simulink model "W06_1_point"  (R2024b)
settings: Solver=ode4  StartTime=0.0  StopTime=T_run  FixedStep=Ts_ctrl  RelTol=1e-3
InitFcn:
  | if ~exist('W06_model_init','file'), addpath(fileparts(get_param('W06_1_point','FileName'))); end, W06_model_init('W06_1_point')
StopFcn:
  | W06_model_done('W06_1_point')
values from neighbouring files (symbols this model uses):
  alloc_prm = [half_beam; l_bow; F_max; F_bow_max]    [W06_setup.m]
  animate = 0    [W06_bow_demo.m]    (also in W06_psi_sweep.m; W06_setup.m = 1)
  beta_c = deg2rad(current_direction)    [W06_setup.m]
  current_speed = 0.0    (= 0)    [W06_setup.m]
  F_bow_max = 250    [W06_setup.m]
  F_max = 500    [W06_setup.m]
  half_beam = 1.027135    [W06_setup.m]
  Kb = Ki_u / Kp_u    (= 0.333333333333)    [W06_setup.m]
  Kd_psi = 200    [W06_setup.m]
  Ki_u = 100    [W06_setup.m]
  Ki_v = 100    [W06_setup.m]
  Kp_psi = 400    [W06_setup.m]
  Kp_u = 300    [W06_setup.m]
  Kp_v = 300    [W06_setup.m]
  Kp_x = 0.4    [W06_setup.m]
  Kp_y = 0.4    [W06_setup.m]
  l_bow = 0.75    [W06_setup.m]
  psi_d = deg2rad(PSI(i))    [W06_psi_sweep.m]    (also in W06_setup.m = deg2rad(hold_deg))
  Ts_ctrl = 0.05    [W06_setup.m]
  u_max = 1.5    [W06_setup.m]
  usv_p = [m_usv; Izz; Xu; Xuu; Yv; Yvv; Nr; Nrr; half_beam; l_bow]    [W06_setup.m]
  v_max = 0.6    [W06_setup.m]
  x0 = [0.1; 0; 0; 0; 0; psi_init]    [W06_setup.m]
  x_d = hold_north    (= 30)    [W06_setup.m]
  y_d = hold_east    (= 20)    [W06_setup.m]
libraries: slpidlib x2
settings Model: Creator=admin  LastModifiedBy=admin

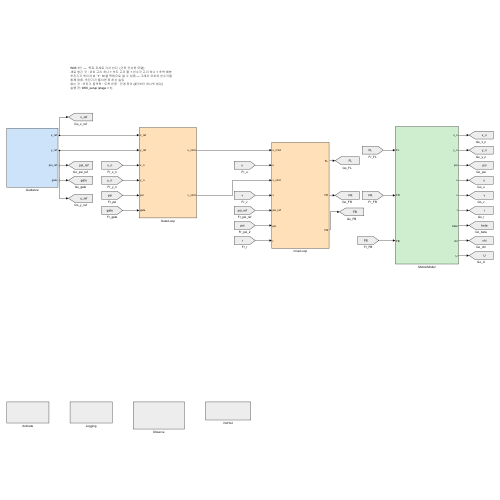
[thumbnail: Simulink's stored preview of the top-level diagram]
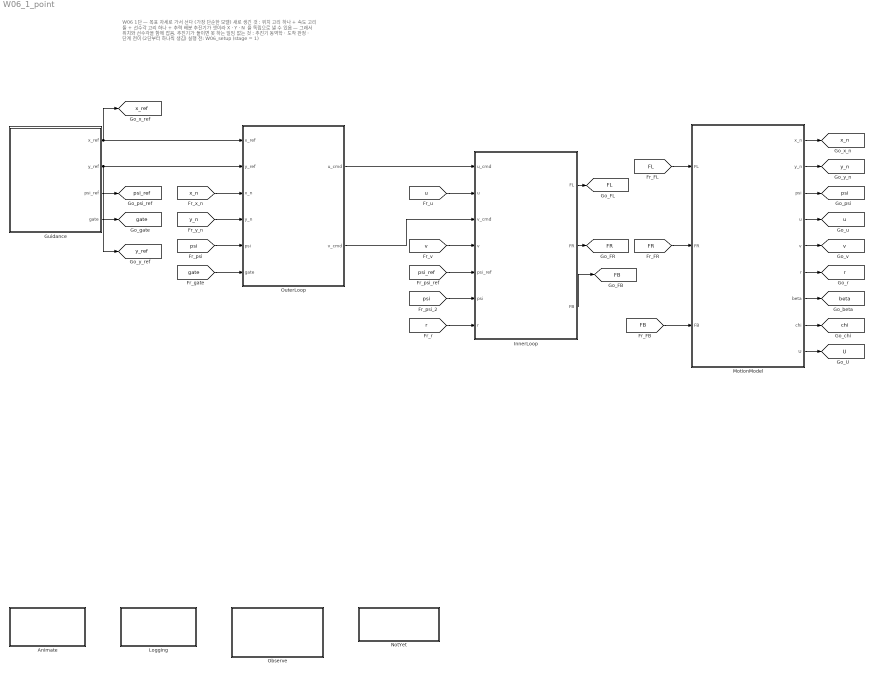
== system W06_1_point ==
  note: W06 1단  —  목표 자세로 가서 선다  (가장 단순한 모델)
      | 새로 생긴 것 : 위치 고리 하나 + 속도 고리 둘 + 선수각 고리 하나 + 추력 배분
      | 추진기가 셋이라 X · Y · N 을 독립으로 낼 수 있음 — 그래서 위치와 선수각을
      | 함께 잡음. 추진기가 둘이면 못 하는 일임
      | 없는 것 : 추진기 동역학 · 도착 판정 · 단계 전이 (2단부터 하나씩 생김)
      | 실행 전: W06_setup (stage = 1)
  Animate : Subsystem
  Guidance : Subsystem
  InnerLoop : Subsystem
  Logging : Subsystem
  MotionModel : Subsystem
  NotYet : Subsystem
  Observe : Subsystem
  OuterLoop : Subsystem
  tag scope: FB=global, FL=global, FR=global, U=global, beta=global, chi=global, gate=global, psi=global, psi_ref=global, r=global, u=global, v=global, x_n=global, x_ref=global, y_n=global, y_ref=global
  wires:
  OuterLoop/2(v_cmd) -> InnerLoop/3(v_cmd)
  OuterLoop/1(u_cmd) -> InnerLoop/1(u_cmd)
  Guidance/1(x_ref) -> OuterLoop/1(x_ref), [x_ref]
  Guidance/2(y_ref) -> OuterLoop/2(y_ref), [y_ref]
  MotionModel/3(psi) -> [psi]
  Guidance/3(psi_ref) -> [psi_ref]
  MotionModel/6(r) -> [r]
  MotionModel/4(u) -> [u]
  MotionModel/5(v) -> [v]
  MotionModel/1(x_n) -> [x_n]
  MotionModel/2(y_n) -> [y_n]
  [FB] -> MotionModel/3(FB)
  [psi] -> InnerLoop/6(psi)
  [psi_ref] -> InnerLoop/5(psi_ref)
  [r] -> InnerLoop/7(r)
  [u] -> InnerLoop/2(u)
  [v] -> InnerLoop/4(v)
  [x_n] -> OuterLoop/3(x_n)
  [y_n] -> OuterLoop/4(y_n)
  MotionModel/9(U) -> [U]
  MotionModel/7(beta) -> [beta]
  MotionModel/8(chi) -> [chi]
  Guidance/4(gate) -> [gate]
  [psi] -> OuterLoop/5(psi)
  [gate] -> OuterLoop/6(gate)
  InnerLoop/3(FB) -> [FB]
  InnerLoop/1(FL) -> [FL]
  InnerLoop/2(FR) -> [FR]
  [FL] -> MotionModel/1(FL)
  [FR] -> MotionModel/2(FR)

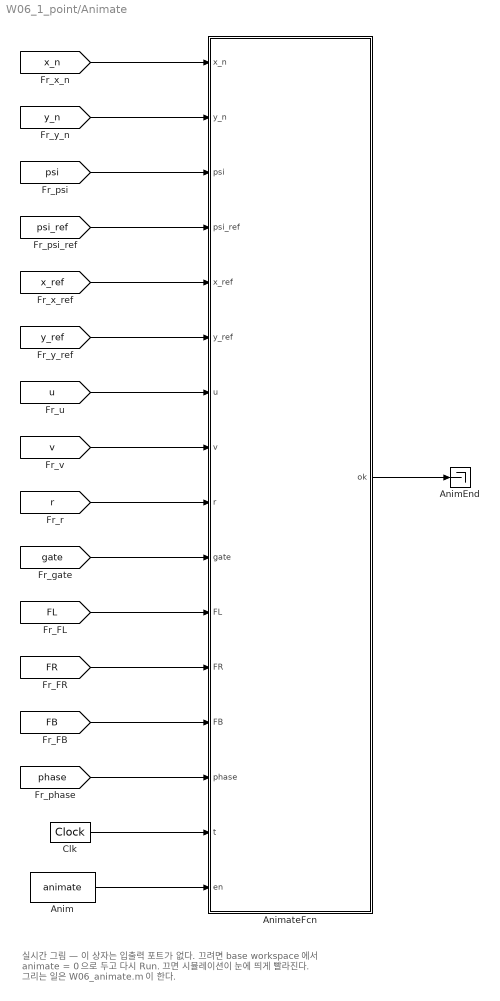
== system W06_1_point/Animate ==
  note: 실시간 그림 — 이 상자는 입출력 포트가 없다.
      | 끄려면 base workspace 에서  animate = 0  으로 두고 다시 Run.
      | 끄면 시뮬레이션이 눈에 띄게 빨라진다.
      | 그리는 일은 W06_animate.m 이 한다.
  Anim : Constant  Value=animate
  AnimEnd : Terminator
  AnimateFcn : MATLAB Function  TreatAsAtomicUnit=on
  Clk : DigitalClock  SampleTime=Ts_ctrl
  wires:
  [x_n] -> AnimateFcn/1(x_n)
  [y_n] -> AnimateFcn/2(y_n)
  [psi] -> AnimateFcn/3(psi)
  [psi_ref] -> AnimateFcn/4(psi_ref)
  [x_ref] -> AnimateFcn/5(x_ref)
  [y_ref] -> AnimateFcn/6(y_ref)
  [u] -> AnimateFcn/7(u)
  [v] -> AnimateFcn/8(v)
  [r] -> AnimateFcn/9(r)
  [gate] -> AnimateFcn/10(gate)
  [FL] -> AnimateFcn/11(FL)
  [FR] -> AnimateFcn/12(FR)
  [FB] -> AnimateFcn/13(FB)
  [phase] -> AnimateFcn/14(phase)
  Clk/1 -> AnimateFcn/15(t)
  Anim/1 -> AnimateFcn/16(en)
  AnimateFcn/1(ok) -> AnimEnd/1

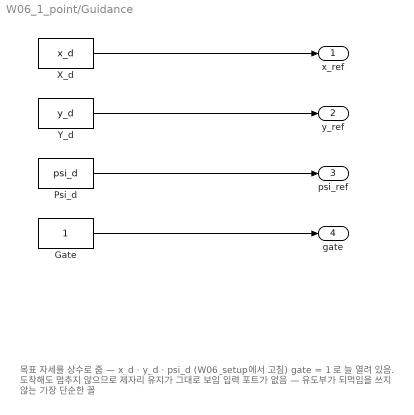
== system W06_1_point/Guidance ==
  note: 목표 자세를 상수로 줌 — x_d · y_d · psi_d (W06_setup 에서 고침)
      | gate = 1 로 늘 열려 있음. 도착해도 멈추지 않으므로 제자리 유지가 그대로 보임
      | 입력 포트가 없음 — 유도부가 되먹임을 쓰지 않는 가장 단순한 꼴
  Gate : Constant
  Psi_d : Constant  Value=psi_d
  X_d : Constant  Value=x_d
  Y_d : Constant  Value=y_d
  x_ref : Outport
  y_ref : Outport  Port=2
  psi_ref : Outport  Port=3
  gate : Outport  Port=4
  wires:
  X_d/1 -> x_ref/1
  Y_d/1 -> y_ref/1
  Psi_d/1 -> psi_ref/1
  Gate/1 -> gate/1

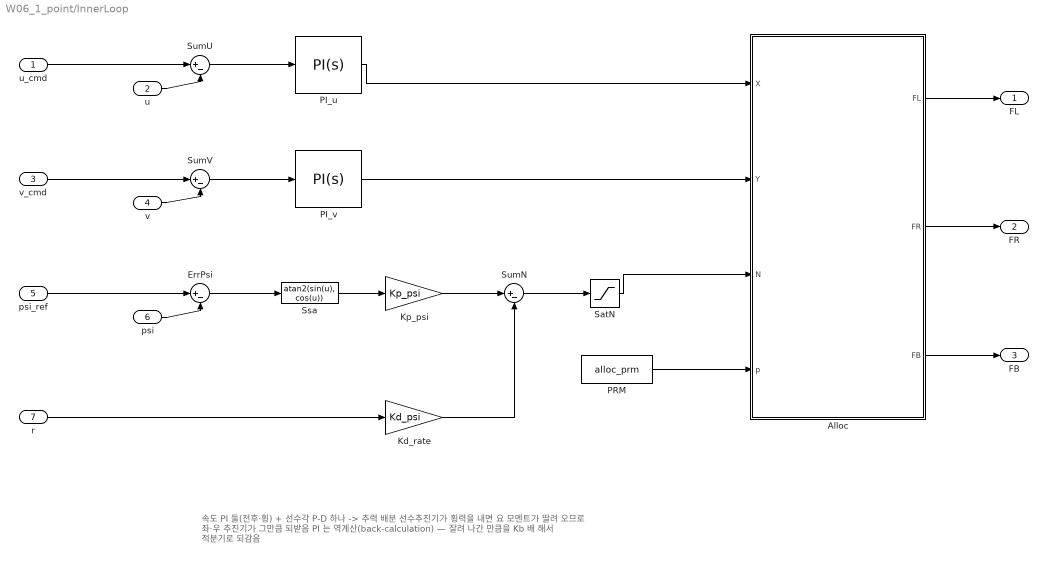
== system W06_1_point/InnerLoop ==
  note: 속도 PI 둘(전후·횡) + 선수각 P-D 하나 -> 추력 배분
      | 선수추진기가 횡력을 내면 요 모멘트가 딸려 오므로 좌·우 추진기가 그만큼 되받음
      | PI 는 역계산(back-calculation) — 잘려 나간 만큼을 Kb 배 해서 적분기로 되감음
  u_cmd : Inport
  u : Inport  Port=2
  v_cmd : Inport  Port=3
  v : Inport  Port=4
  psi_ref : Inport  Port=5
  psi : Inport  Port=6
  r : Inport  Port=7
  Alloc : MATLAB Function  TreatAsAtomicUnit=on
  ErrPsi : Sum  Inputs=|+-
  Kd_rate : Gain  Gain=Kd_psi
  Kp_psi : Gain  Gain=Kp_psi
  PI_u : slpidlib/PID Controller  Controller=PI  Form=Parallel  TimeDomain=Continuous-time  UseExternalTs=off  SampleTime=-1  IntegratorMethod=Forward Euler  FilterMethod=Forward Euler  ControllerParametersSource=internal  P=Kp_u  I=Ki_u  UseKiTs=off  D=0  UseExternalDerivativeSource=off  N=100  UseFilter=on  TunerSelectOption=Transfer Function Based (PID Tuner App)  InitialConditionSource=internal  InitialConditionForIntegrator=0  InitialConditionForFilter=0  DifferentiatorICPrevScaledInput=0  ExternalReset=none  TrackingMode=off  Kt=1  LimitOutput=on  SatLimitsSource=internal  UpperSaturationLimit=2*F_max  LowerSaturationLimit=-(2*F_max)  LinearizeAsGain=on  AntiWindupMode=back-calculation  Kb=Kb  LimitIntegrator=off  UpperIntegratorSaturationLimit=inf  LowerIntegratorSaturationLimit=-inf  POutMin=[]  POutMax=[]  IOutMin=[]  IOutMax=[]  DOutMin=[]  DOutMax=[]  NOutMin=[]  NOutMax=[]  SumOutMin=[]  SumOutMax=[]  SaturationOutMin=[]  SaturationOutMax=[]  PParamMin=[]  PParamMax=[]  IParamMin=[]  IParamMax=[]  DParamMin=[]  DParamMax=[]  NParamMin=[]  NParamMax=[]  KbParamMin=[]  KbParamMax=[]  KtParamMin=[]  KtParamMax=[]  KbOutMin=[]  KbOutMax=[]  KtOutMin=[]  KtOutMax=[]  IntegratorOutMin=[]  IntegratorOutMax=[]  FilterOutMin=[]  FilterOutMax=[]  SumI1OutMin=[]  SumI1OutMax=[]  SumI2OutMin=[]  SumI2OutMax=[]  SumI3OutMin=[]  SumI3OutMax=[]  SumI4OutMin=[]  SumI4OutMax=[]  SumDOutMin=[]  SumDOutMax=[]  DifferentiatorOutMin=[]  DifferentiatorOutMax=[]  FilterDiffOutCoefMin=[]  FilterDiffOutCoefMax=[]  ReciprocalOutMin=[]  ReciprocalOutMax=[]  SumDenOutMin=[]  SumDenOutMax=[]  SumNumOutMin=[]  SumNumOutMax=[]  DivideOutMin=[]  DivideOutMax=[]  UdiffTsProdOutMin=[]  UdiffTsProdOutMax=[]  NTsProdOutMin=[]  NTsProdOutMax=[]  UintegralTsProdOutMin=[]  UintegralTsProdOutMax=[]  UngainTsProdOutMin=[]  UngainTsProdOutMax=[]  ClampingZeroOutDataTypeStr=Inherit: Inherit via back propagation  ClampingZeroOutMin=[]  ClampingZeroOutMax=[]  FilterDenConstantOutDataTypeStr=Inherit: Inherit via back propagation  FilterDenConstantOutMin=[]  FilterDenConstantOutMax=[]  PCopyOutDataTypeStr=Inherit: Inherit via back propagation  PCopyOutMin=[]  PCopyOutMax=[]  NCopyOutDataTypeStr=Inherit: Inherit via back propagation  NCopyOutMin=[]  NCopyOutMax=[]  IntegratorContinuousStateAttributes=''  IntegratorStateMustResolveToSignalObject=off  IntegratorRTWStateStorageClass=Auto  FilterContinuousStateAttributes=''  FilterStateMustResolveToSignalObject=off  FilterRTWStateStorageClass=Auto  ParallelPVariant=InternalParameters  IdealPVariant=Disabled  IVariant=InternalParameters  DVariant=Disabled  IntegratorVariant=Continuous  SatVariant=Enabled  AWVariant=BackCalculation  PCopyVariant=Disabled  TRVariant=Disabled  FdbkBlocksVariant=Forward  IdealPFdbkVariant=Disabled  SatFdbkVariant=Disabled  DerivativeFilterVariant=Disabled  NVariant=Disabled  NCopyVariant=Disabled_SignalSpec  FilterICVariant=Disabled  IntegratorICVariant=InternalICs  ExternalResetVariant=Disabled  TRSumVariant=Passthrough  SumFdbkVariant=Disabled  SumVariant=Sum_PI  TsampFilterVariant=InternalTs  TsampNgainVariant=Passthrough  TsampIntegralVariant=Disabled_SignalSpec  ExternalSaturationOutDataTypeStr=Inherit: Same as second input  DerivativeSourceVariant=Disabled  PreIntVariant=InternalPreInt
  PI_v : slpidlib/PID Controller  Controller=PI  Form=Parallel  TimeDomain=Continuous-time  UseExternalTs=off  SampleTime=-1  IntegratorMethod=Forward Euler  FilterMethod=Forward Euler  ControllerParametersSource=internal  P=Kp_v  I=Ki_v  UseKiTs=off  D=0  UseExternalDerivativeSource=off  N=100  UseFilter=on  TunerSelectOption=Transfer Function Based (PID Tuner App)  InitialConditionSource=internal  InitialConditionForIntegrator=0  InitialConditionForFilter=0  DifferentiatorICPrevScaledInput=0  ExternalReset=none  TrackingMode=off  Kt=1  LimitOutput=on  SatLimitsSource=internal  UpperSaturationLimit=F_bow_max  LowerSaturationLimit=-(F_bow_max)  LinearizeAsGain=on  AntiWindupMode=back-calculation  Kb=Kb  LimitIntegrator=off  UpperIntegratorSaturationLimit=inf  LowerIntegratorSaturationLimit=-inf  POutMin=[]  POutMax=[]  IOutMin=[]  IOutMax=[]  DOutMin=[]  DOutMax=[]  NOutMin=[]  NOutMax=[]  SumOutMin=[]  SumOutMax=[]  SaturationOutMin=[]  SaturationOutMax=[]  PParamMin=[]  PParamMax=[]  IParamMin=[]  IParamMax=[]  DParamMin=[]  DParamMax=[]  NParamMin=[]  NParamMax=[]  KbParamMin=[]  KbParamMax=[]  KtParamMin=[]  KtParamMax=[]  KbOutMin=[]  KbOutMax=[]  KtOutMin=[]  KtOutMax=[]  IntegratorOutMin=[]  IntegratorOutMax=[]  FilterOutMin=[]  FilterOutMax=[]  SumI1OutMin=[]  SumI1OutMax=[]  SumI2OutMin=[]  SumI2OutMax=[]  SumI3OutMin=[]  SumI3OutMax=[]  SumI4OutMin=[]  SumI4OutMax=[]  SumDOutMin=[]  SumDOutMax=[]  DifferentiatorOutMin=[]  DifferentiatorOutMax=[]  FilterDiffOutCoefMin=[]  FilterDiffOutCoefMax=[]  ReciprocalOutMin=[]  ReciprocalOutMax=[]  SumDenOutMin=[]  SumDenOutMax=[]  SumNumOutMin=[]  SumNumOutMax=[]  DivideOutMin=[]  DivideOutMax=[]  UdiffTsProdOutMin=[]  UdiffTsProdOutMax=[]  NTsProdOutMin=[]  NTsProdOutMax=[]  UintegralTsProdOutMin=[]  UintegralTsProdOutMax=[]  UngainTsProdOutMin=[]  UngainTsProdOutMax=[]  ClampingZeroOutDataTypeStr=Inherit: Inherit via back propagation  ClampingZeroOutMin=[]  ClampingZeroOutMax=[]  FilterDenConstantOutDataTypeStr=Inherit: Inherit via back propagation  FilterDenConstantOutMin=[]  FilterDenConstantOutMax=[]  PCopyOutDataTypeStr=Inherit: Inherit via back propagation  PCopyOutMin=[]  PCopyOutMax=[]  NCopyOutDataTypeStr=Inherit: Inherit via back propagation  NCopyOutMin=[]  NCopyOutMax=[]  IntegratorContinuousStateAttributes=''  IntegratorStateMustResolveToSignalObject=off  IntegratorRTWStateStorageClass=Auto  FilterContinuousStateAttributes=''  FilterStateMustResolveToSignalObject=off  FilterRTWStateStorageClass=Auto  ParallelPVariant=InternalParameters  IdealPVariant=Disabled  IVariant=InternalParameters  DVariant=Disabled  IntegratorVariant=Continuous  SatVariant=Enabled  AWVariant=BackCalculation  PCopyVariant=Disabled  TRVariant=Disabled  FdbkBlocksVariant=Forward  IdealPFdbkVariant=Disabled  SatFdbkVariant=Disabled  DerivativeFilterVariant=Disabled  NVariant=Disabled  NCopyVariant=Disabled_SignalSpec  FilterICVariant=Disabled  IntegratorICVariant=InternalICs  ExternalResetVariant=Disabled  TRSumVariant=Passthrough  SumFdbkVariant=Disabled  SumVariant=Sum_PI  TsampFilterVariant=InternalTs  TsampNgainVariant=Passthrough  TsampIntegralVariant=Disabled_SignalSpec  ExternalSaturationOutDataTypeStr=Inherit: Same as second input  DerivativeSourceVariant=Disabled  PreIntVariant=InternalPreInt
  PRM : Constant  Value=alloc_prm
  SatN : Saturate  UpperLimit=2*F_max*half_beam + F_bow_max*l_bow  LowerLimit=-(2*F_max*half_beam + F_bow_max*l_bow)
  Ssa : Fcn  Expr=atan2(sin(u), cos(u))
  SumN : Sum  Inputs=|+-
  SumU : Sum  Inputs=|+-
  SumV : Sum  Inputs=|+-
  FL : Outport
  FR : Outport  Port=2
  FB : Outport  Port=3
  wires:
  u_cmd/1 -> SumU/1
  u/1 -> SumU/2
  v_cmd/1 -> SumV/1
  v/1 -> SumV/2
  SumU/1 -> PI_u/1
  SumV/1 -> PI_v/1
  ErrPsi/1 -> Ssa/1
  psi_ref/1 -> ErrPsi/1
  psi/1 -> ErrPsi/2
  Ssa/1 -> Kp_psi/1
  r/1 -> Kd_rate/1
  Kp_psi/1 -> SumN/1
  Kd_rate/1 -> SumN/2
  SumN/1 -> SatN/1
  PI_u/1 -> Alloc/1(X)
  PI_v/1 -> Alloc/2(Y)
  SatN/1 -> Alloc/3(N)
  PRM/1 -> Alloc/4(p)
  Alloc/1(FL) -> FL/1
  Alloc/2(FR) -> FR/1
  Alloc/3(FB) -> FB/1

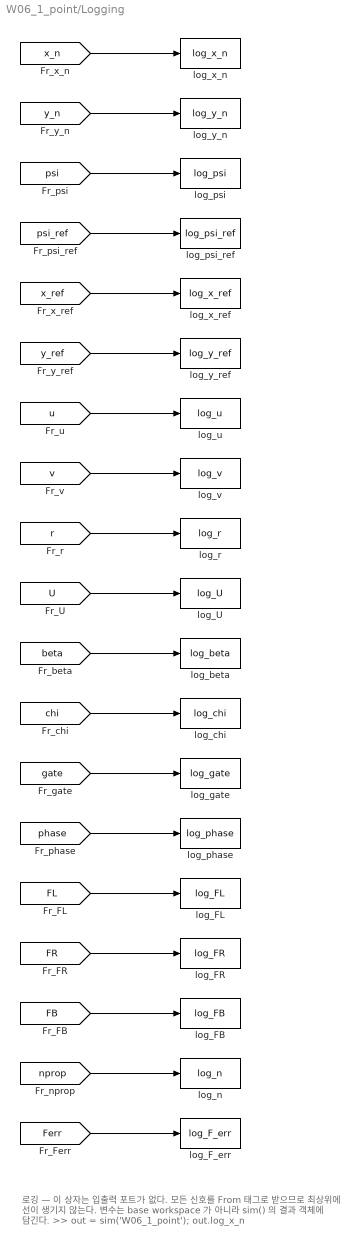
== system W06_1_point/Logging ==
  note: 로깅 — 이 상자는 입출력 포트가 없다.
      | 모든 신호를 From 태그로 받으므로 최상위에 선이 생기지 않는다.
      | 변수는 base workspace 가 아니라 sim() 의 결과 객체에 담긴다.
      |   >> out = sim('W06_1_point');  out.log_x_n
  log_FB : ToWorkspace  VariableName=log_FB  SaveFormat=Timeseries  SampleTime=Ts_ctrl
  log_FL : ToWorkspace  VariableName=log_FL  SaveFormat=Timeseries  SampleTime=Ts_ctrl
  log_FR : ToWorkspace  VariableName=log_FR  SaveFormat=Timeseries  SampleTime=Ts_ctrl
  log_F_err : ToWorkspace  VariableName=log_F_err  SaveFormat=Timeseries  SampleTime=Ts_ctrl
  log_U : ToWorkspace  VariableName=log_U  SaveFormat=Timeseries  SampleTime=Ts_ctrl
  log_beta : ToWorkspace  VariableName=log_beta  SaveFormat=Timeseries  SampleTime=Ts_ctrl
  log_chi : ToWorkspace  VariableName=log_chi  SaveFormat=Timeseries  SampleTime=Ts_ctrl
  log_gate : ToWorkspace  VariableName=log_gate  SaveFormat=Timeseries  SampleTime=Ts_ctrl
  log_n : ToWorkspace  VariableName=log_n  SaveFormat=Timeseries  SampleTime=Ts_ctrl
  log_phase : ToWorkspace  VariableName=log_phase  SaveFormat=Timeseries  SampleTime=Ts_ctrl
  log_psi : ToWorkspace  VariableName=log_psi  SaveFormat=Timeseries  SampleTime=Ts_ctrl
  log_psi_ref : ToWorkspace  VariableName=log_psi_ref  SaveFormat=Timeseries  SampleTime=Ts_ctrl
  log_r : ToWorkspace  VariableName=log_r  SaveFormat=Timeseries  SampleTime=Ts_ctrl
  log_u : ToWorkspace  VariableName=log_u  SaveFormat=Timeseries  SampleTime=Ts_ctrl
  log_v : ToWorkspace  VariableName=log_v  SaveFormat=Timeseries  SampleTime=Ts_ctrl
  log_x_n : ToWorkspace  VariableName=log_x_n  SaveFormat=Timeseries  SampleTime=Ts_ctrl
  log_x_ref : ToWorkspace  VariableName=log_x_ref  SaveFormat=Timeseries  SampleTime=Ts_ctrl
  log_y_n : ToWorkspace  VariableName=log_y_n  SaveFormat=Timeseries  SampleTime=Ts_ctrl
  log_y_ref : ToWorkspace  VariableName=log_y_ref  SaveFormat=Timeseries  SampleTime=Ts_ctrl
  wires:
  [x_n] -> log_x_n/1
  [y_n] -> log_y_n/1
  [psi] -> log_psi/1
  [psi_ref] -> log_psi_ref/1
  [x_ref] -> log_x_ref/1
  [y_ref] -> log_y_ref/1
  [u] -> log_u/1
  [v] -> log_v/1
  [r] -> log_r/1
  [U] -> log_U/1
  [beta] -> log_beta/1
  [chi] -> log_chi/1
  [gate] -> log_gate/1
  [phase] -> log_phase/1
  [FL] -> log_FL/1
  [FR] -> log_FR/1
  [FB] -> log_FB/1
  [nprop] -> log_n/1
  [Ferr] -> log_F_err/1

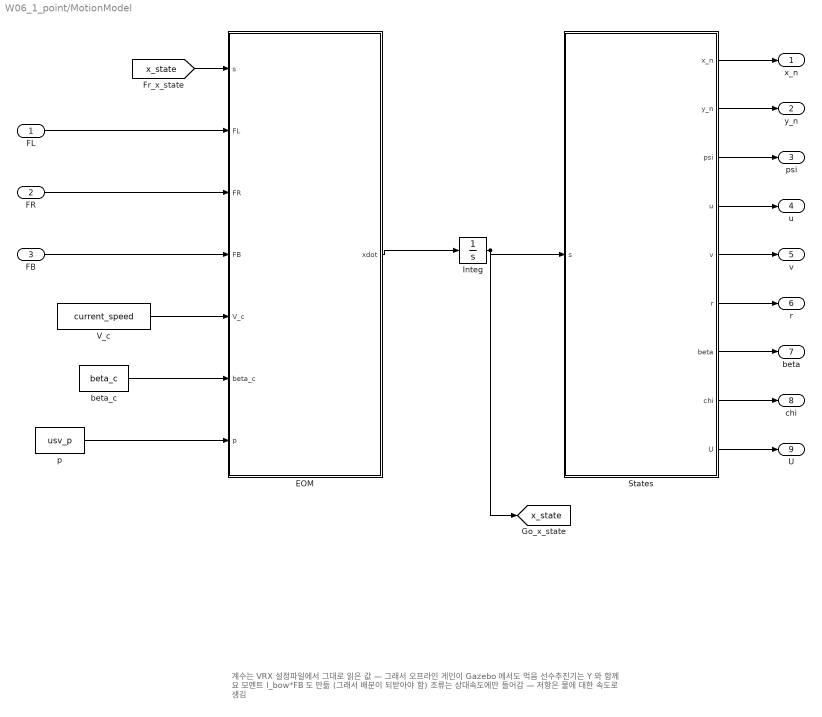
== system W06_1_point/MotionModel ==
  note: 계수는 VRX 설정파일에서 그대로 읽은 값 — 그래서 오프라인 게인이 Gazebo 에서도 먹음
      | 선수추진기는 Y 와 함께 요 모멘트 l_bow*FB 도 만듦 (그래서 배분이 되받아야 함)
      | 조류는 상대속도에만 들어감 — 저항은 물에 대한 속도로 생김
  FL : Inport
  FR : Inport  Port=2
  FB : Inport  Port=3
  EOM : MATLAB Function  TreatAsAtomicUnit=on
  Integ : Integrator  InitialCondition=x0
  States : MATLAB Function  TreatAsAtomicUnit=on
  V_c : Constant  Value=current_speed
  beta_c : Constant  Value=beta_c
  p : Constant  Value=usv_p
  x_n : Outport
  y_n : Outport  Port=2
  psi : Outport  Port=3
  u : Outport  Port=4
  v : Outport  Port=5
  r : Outport  Port=6
  beta : Outport  Port=7
  chi : Outport  Port=8
  U : Outport  Port=9
  tag scope: x_state=global
  wires:
  FL/1 -> EOM/2(FL)
  FR/1 -> EOM/3(FR)
  FB/1 -> EOM/4(FB)
  V_c/1 -> EOM/5(V_c)
  beta_c/1 -> EOM/6(beta_c)
  p/1 -> EOM/7(p)
  EOM/1(xdot) -> Integ/1
  Integ/1 -> States/1(s), [x_state]
  [x_state] -> EOM/1(s)
  States/1(x_n) -> x_n/1
  States/2(y_n) -> y_n/1
  States/3(psi) -> psi/1
  States/4(u) -> u/1
  States/5(v) -> v/1
  States/6(r) -> r/1
  States/7(beta) -> beta/1
  States/8(chi) -> chi/1
  States/9(U) -> U/1

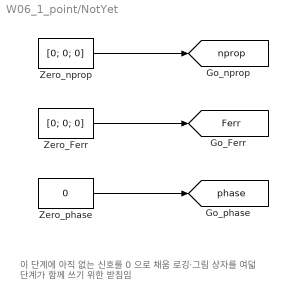
== system W06_1_point/NotYet ==
  note: 이 단계에 아직 없는 신호를 0 으로 채움
      | 로깅·그림 상자를 여덟 단계가 함께 쓰기 위한 받침임
  Zero_Ferr : Constant  Value=[0; 0; 0]
  Zero_nprop : Constant  Value=[0; 0; 0]
  Zero_phase : Constant  Value=0
  tag scope: Ferr=global, nprop=global, phase=global
  wires:
  Zero_nprop/1 -> [nprop]
  Zero_Ferr/1 -> [Ferr]
  Zero_phase/1 -> [phase]

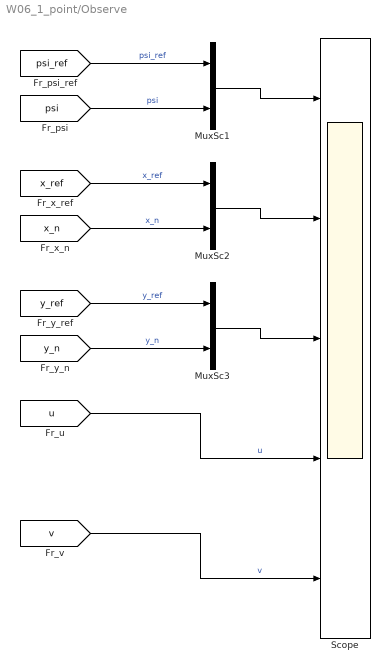
== system W06_1_point/Observe ==
  MuxSc1 : Mux  Inputs=2
  MuxSc2 : Mux  Inputs=2
  MuxSc3 : Mux  Inputs=2
  Scope : Scope  NumInputPorts=5
  wires:
  [psi_ref] -> MuxSc1/1  "psi_ref"
  [psi] -> MuxSc1/2  "psi"
  MuxSc1/1 -> Scope/1
  [x_ref] -> MuxSc2/1  "x_ref"
  [x_n] -> MuxSc2/2  "x_n"
  MuxSc2/1 -> Scope/2
  [y_ref] -> MuxSc3/1  "y_ref"
  [y_n] -> MuxSc3/2  "y_n"
  MuxSc3/1 -> Scope/3
  [u] -> Scope/4  "u"
  [v] -> Scope/5  "v"

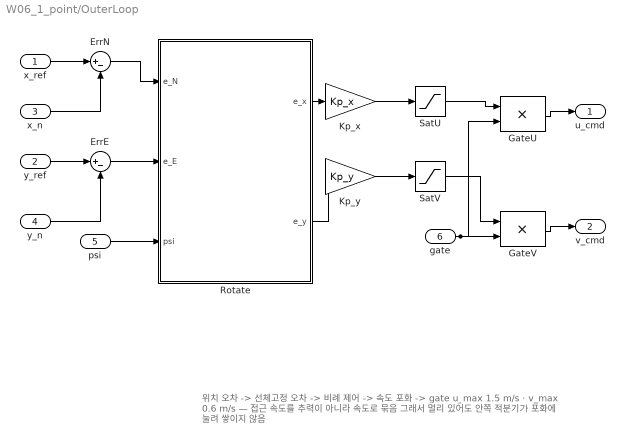
== system W06_1_point/OuterLoop ==
  note: 위치 오차 -> 선체고정 오차 -> 비례 제어 -> 속도 포화 -> gate
      | u_max 1.5 m/s · v_max 0.6 m/s — 접근 속도를 추력이 아니라 속도로 묶음
      | 그래서 멀리 있어도 안쪽 적분기가 포화에 눌려 쌓이지 않음
  x_ref : Inport
  y_ref : Inport  Port=2
  x_n : Inport  Port=3
  y_n : Inport  Port=4
  psi : Inport  Port=5
  gate : Inport  Port=6
  ErrE : Sum  Inputs=|+-
  ErrN : Sum  Inputs=|+-
  GateU : Product
  GateV : Product
  Kp_x : Gain  Gain=Kp_x
  Kp_y : Gain  Gain=Kp_y
  Rotate : MATLAB Function  TreatAsAtomicUnit=on
  SatU : Saturate  UpperLimit=u_max  LowerLimit=-(u_max)
  SatV : Saturate  UpperLimit=v_max  LowerLimit=-(v_max)
  u_cmd : Outport
  v_cmd : Outport  Port=2
  wires:
  psi/1 -> Rotate/3(psi)
  ErrE/1 -> Rotate/2(e_E)
  x_ref/1 -> ErrN/1
  ErrN/1 -> Rotate/1(e_N)
  x_n/1 -> ErrN/2
  y_ref/1 -> ErrE/1
  y_n/1 -> ErrE/2
  Rotate/1(e_x) -> Kp_x/1
  Rotate/2(e_y) -> Kp_y/1
  Kp_x/1 -> SatU/1
  Kp_y/1 -> SatV/1
  SatU/1 -> GateU/1
  SatV/1 -> GateV/1
  gate/1 -> GateV/2, GateU/2
  GateU/1 -> u_cmd/1
  GateV/1 -> v_cmd/1

== matlab function W06_1_point/InnerLoop/Alloc ==
  data: X input; FL output; Y input; N input; p input; FR output; FB output
function [FL, FR, FB] = Alloc(X, Y, N, p)
%#codegen
%  추력 배분 — 요구 힘·모멘트를 세 추진기로 나눈다.
%
%    X = FL + FR                      전후력 [N]
%    Y = FB                           횡력 [N]  — 선수추진기만 낸다
%    N = (FL - FR)*b + l3*FB          요 모멘트 [N m]
%
%  p = [b; l3; Fmax; Fbmax]
%    b     half_beam   좌·우 추진기까지의 반폭 [m]
%    l3    l_bow       무게중심에서 선수추진기까지 [m]
%    Fmax  선미 추진기 추력 한계 [N],  Fbmax 선수추진기 추력 한계 [N]
%
%  선수추진기가 횡력을 내면 요 모멘트 l3*FB 가 딸려 온다. 그것을 좌·우
%  추진기가 되받아 빼야 선수각이 돌아가지 않는다 — 아래 N - l3*FB 가 그것이다.
b = p(1);  l3 = p(2);  Fmax = p(3);  Fbmax = p(4);
FB = Y;
if FB >  Fbmax, FB =  Fbmax; end
if FB < -Fbmax, FB = -Fbmax; end
%  포화된 뒤의 FB 로 모멘트를 센다 — 실제로 딸려 온 만큼만 되받는다
M  = N - l3*FB;
FL = X/2 + M/(2*b);
FR = X/2 - M/(2*b);
if FL >  Fmax, FL =  Fmax; end
if FL < -Fmax, FL = -Fmax; end
if FR >  Fmax, FR =  Fmax; end
if FR < -Fmax, FR = -Fmax; end

== matlab function W06_1_point/OuterLoop/Rotate ==
  data: e_N input; e_x output; e_E input; psi input; e_y output
function [e_x, e_y] = Rotate(e_N, e_E, psi)
%#codegen
%  NED 위치 오차를 선체고정 오차로 돌린다. e_x 앞쪽, e_y 우현쪽 [m]
e_x =  cos(psi)*e_N + sin(psi)*e_E;
e_y = -sin(psi)*e_N + cos(psi)*e_E;

== matlab function W06_1_point/MotionModel/EOM ==
  data: s input; xdot output; FL input; FR input; FB input; V_c input; beta_c input; p input
function xdot = EOM(s, FL, FR, FB, V_c, beta_c, p)
%#codegen
%  3자유도 운동방정식.  s = [u v r x_n y_n psi]'
%
%    조류는 상대속도에만 들어간다 — 저항은 물에 대한 속도로 생긴다
%    부가질량은 0 으로 둔다 (VRX 설정도 0 이다)
u = s(1);  v = s(2);  r = s(3);  psi = s(6);
m_s  = p(1);  Izz = p(2);
Xu   = p(3);  Xuu = p(4);
Yv   = p(5);  Yvv = p(6);
Nr   = p(7);  Nrr = p(8);
b_h  = p(9);  l3  = p(10);

%  조류를 선체좌표로 — 물에 대한 상대속도 u_r, v_r
u_c = V_c*cos(beta_c - psi);
v_c = V_c*sin(beta_c - psi);
u_r = u - u_c;
v_r = v - v_c;

%  추진기가 내는 힘과 모멘트
X = FL + FR;
Y = FB;
N = (FL - FR)*b_h + l3*FB;

%  저항 — 선형 + 제곱 (제곱항이 있어 속도가 커질수록 빨리 늘어난다)
Dx = (Xu + Xuu*abs(u_r))*u_r;
Dy = (Yv + Yvv*abs(v_r))*v_r;
Dn = (Nr + Nrr*abs(r))*r;

%  v*r, -u*r 은 좌표계가 함께 돌기 때문에 생기는 항이다
du = (X - Dx)/m_s + v*r;
dv = (Y - Dy)/m_s - u*r;
dr = (N - Dn)/Izz;

%  선체속도를 NED 로 — 이것이 위치의 미분이다
xdot = [du; dv; dr; ...
        u*cos(psi) - v*sin(psi); ...
        u*sin(psi) + v*cos(psi); ...
        r];

== matlab function W06_1_point/MotionModel/States ==
  data: s input; x_n output; y_n output; psi output; u output; v output; r output; beta output; chi output; U output
function [x_n, y_n, psi, u, v, r, beta, chi, U] = States(s)
%#codegen
%  상태벡터를 쓰기 좋은 이름으로 풀어 놓는다.
%    U    대지속력 [m/s]
%    beta 크랩각 — 뱃머리와 실제 가는 방향의 차이 [rad]
%    chi  침로 = psi + beta, 실제 가는 방향 [rad]
u = s(1);  v = s(2);  r = s(3);
x_n = s(4);  y_n = s(5);  psi = s(6);
U = sqrt(u*u + v*v);
beta = atan2(v, u);
c = psi + beta;
chi = atan2(sin(c), cos(c));

== matlab function W06_1_point/Animate/AnimateFcn ==
  data: x_n input; y_n input; psi input; psi_ref input; x_ref input; y_ref input; u input; ok output; v input; r input; gate input; FL input; FR input; FB input; phase input; t input; en input
function ok = AnimateFcn(x_n, y_n, psi, psi_ref, x_ref, y_ref, u, v, r, gate, FL, FR, FB, phase, t, en)
%#codegen
% Live plot while the model runs. A MATLAB Function block cannot
% plot, so the drawing function is declared extrinsic: Simulink
% calls plain MATLAB instead of generating code for it.
coder.extrinsic('W06_animate');
ok = 1;
if en > 0.5
    W06_animate(x_n, y_n, psi, psi_ref, x_ref, y_ref, u, v, r, gate, FL, FR, FB, phase, t);
end
